simulink library "lib_SecCtrl_MASmsg"  (R2026a)
settings: Solver=VariableStepAuto
undefined symbols (not defined in the file): buses_lf, DiscIntNeverNeededParam, entity, iPs_lf, iQs_lf, last_send, m, Ps_lf, Qs_lf, set_DG_up, set_extra_satur, set_sending_cost, v_buses_mod
libraries: simulink x400, sl_discontinuities x10, eeGeneralControl x5
(part 4 of 12)

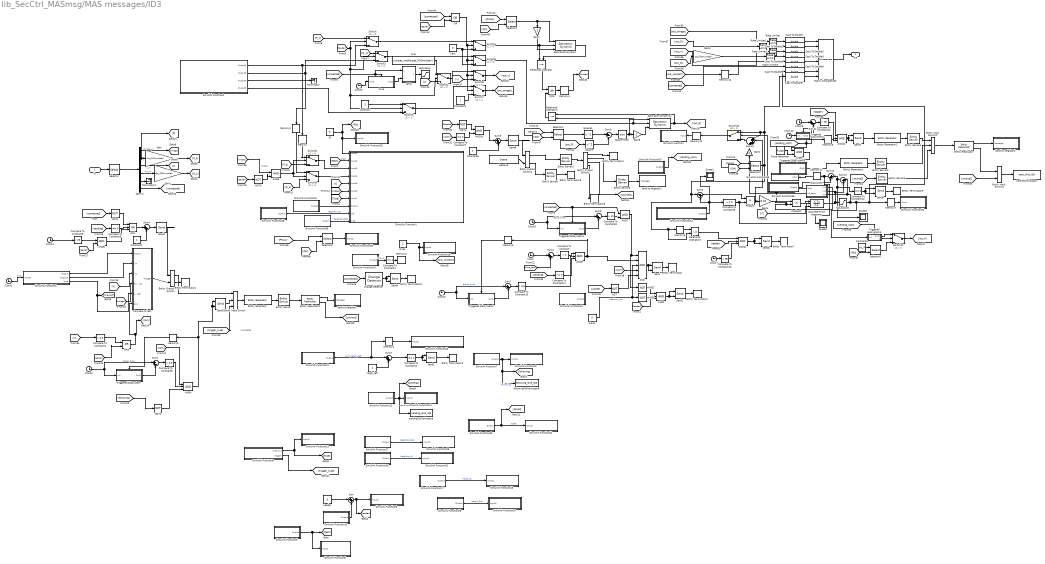
== system lib_SecCtrl_MASmsg/MAS messages/ID3 ==
  note: Variables
  in : Inport
  AND : Logic  Inputs=5  IconShape=distinctive  AllPortsSameDT=off  OutDataTypeStr=boolean
  AND{1,3..4,11..12} (5 alike) : Logic  Inputs=3  IconShape=distinctive  AllPortsSameDT=off  OutDataTypeStr=boolean
  AND{5..7,9..10} (5 alike) : Logic  IconShape=distinctive  AllPortsSameDT=off  OutDataTypeStr=boolean
  AND2 : Logic  Operator=NOT  IconShape=distinctive  AllPortsSameDT=off  OutDataTypeStr=boolean
  AND8 : Logic  Operator=NOT  IconShape=distinctive  AllPortsSameDT=off  OutDataTypeStr=boolean
  Cast To Double{,1..7} (8 alike) : DataTypeConversion  OutDataTypeStr=double  SaturateOnIntegerOverflow=off  RndMeth=Floor
  Change Detector : eeGeneralControl/Change Detector  VariantControl=Variant1  LabelModeActiveChoice=Discrete  ChangeType=Falling edge  x0=0  Ts=-1
  Clock{,1..8,10} (10 alike) : Clock
  Compare To Constant : simulink/Logic and Bit Operations/Compare To Constant  relop=>  const=2  OutDataTypeStr=boolean  ZeroCross=off
  Compare To Constant1 : simulink/Logic and Bit Operations/Compare To Constant  relop===  const=1  OutDataTypeStr=boolean  ZeroCross=off
  Compare To Constant10 : simulink/Logic and Bit Operations/Compare To Constant  relop=>  const=0.5  OutDataTypeStr=boolean  ZeroCross=off
  Compare To Constant11 : simulink/Logic and Bit Operations/Compare To Constant  relop=~=  const=0  OutDataTypeStr=uint8  ZeroCross=off
  Compare To Constant12 : simulink/Logic and Bit Operations/Compare To Constant  relop=>  const=90  OutDataTypeStr=boolean
  Compare To Constant13 : simulink/Logic and Bit Operations/Compare To Constant  relop=>  const=95  OutDataTypeStr=boolean
  Compare To Constant14 : simulink/Logic and Bit Operations/Compare To Constant  relop===  const=0  OutDataTypeStr=boolean
  Compare To Constant2 : simulink/Logic and Bit Operations/Compare To Constant  relop===  const=0  OutDataTypeStr=boolean  ZeroCross=off
  Compare To Constant3 : simulink/Logic and Bit Operations/Compare To Constant  relop===  const=0  OutDataTypeStr=uint8  ZeroCross=off
  Compare To Constant4 : simulink/Logic and Bit Operations/Compare To Constant  relop=>  const=0.5  OutDataTypeStr=boolean  ZeroCross=off
  Compare To Constant5 : simulink/Logic and Bit Operations/Compare To Constant  relop=>  const=0.5  OutDataTypeStr=boolean  ZeroCross=off
  Compare To Constant6 : simulink/Logic and Bit Operations/Compare To Constant  relop=<  const=25  OutDataTypeStr=boolean  ZeroCross=off
  Compare To Constant7 : simulink/Logic and Bit Operations/Compare To Constant  relop===  const=0  OutDataTypeStr=uint8  ZeroCross=off
  Compare To Constant8 : simulink/Logic and Bit Operations/Compare To Constant  relop=>  const=10  OutDataTypeStr=boolean  ZeroCross=off
  Compare To Constant9 : simulink/Logic and Bit Operations/Compare To Constant  relop=~=  const=0  OutDataTypeStr=boolean
  Compare to last : Subsystem
  Constant{,1..2,6} (4 alike) : Constant
  Constant3 : Constant  Value=Ps_lf  VectorParams1D=off
  Demux : Demux  Outputs=6
  Discrete-Time Integrator : DiscreteIntegrator  ExternalReset=rising  InitialConditionSource=external  ICPrevOutput=DiscIntNeverNeededParam  ICPrevScaledInput=DiscIntNeverNeededParam
  Entity Input Switch : EntityInputSwitch  InputPortMessageModes=m,m,m  OutputPortMessageModes=m  NumberInputPorts=3
      settings: InputPortMap=u1,u2,u3
  Entity Input Switch1 : EntityInputSwitch  InputPortMessageModes=m,m  OutputPortMessageModes=m
  Entity Input Switch2 : EntityInputSwitch  InputPortMessageModes=m,m,m  OutputPortMessageModes=m  NumberInputPorts=3
      settings: InputPortMap=u1,u2,u3
  Entity Output Switch : EntityOutputSwitch  InputPortMessageModes=m,m  OutputPortMessageModes=m,m  SwitchingCriterion=From control port  SwitchAttributeName=Attribute1
      settings: InputPortMap=u0,u1
  Entity Output Switch1 : EntityOutputSwitch  InputPortMessageModes=m,m  OutputPortMessageModes=m,m  SwitchingCriterion=From control port  SwitchAttributeName=Attribute1
      settings: InputPortMap=u0,u1
  Entity Output Switch2 : EntityOutputSwitch  InputPortMessageModes=m  OutputPortMessageModes=m,m,m,m  NumberOutputPorts=4  SwitchingCriterion=From attribute  SwitchAttributeName=Select
      settings: OutputPortMap=o0,o1,o2,o3
  Entity Generator : EntityGenerator  InputPortMessageModes=m  OutputPortMessageModes=m  GenerationMethod=Event-based  Period=0.01  AttributeName=DG_up|Source|Dest|P_s|Q_s|v|omega|Opt|type|Select|Neighbor_ID|Neighbor_Opt  AttributeInitialValue=0|0|0|0|0|0|0|1|0|0|1|1  EntityType=Structured  EntityTypeName=Message
      settings: InputPortMap=u0
  Entity Generator1 : EntityGenerator  InputPortMessageModes=m  OutputPortMessageModes=m  GenerationMethod=Event-based  TimeSource=Signal port  Period=0.1  GenerateEntityAtSimulationStart=off  AttributeName=DG_up|Source|Dest|P_s|Q_s|v|omega|Opt|type|Select|Neighbor_ID|Neighbor_Opt  AttributeInitialValue=0|0|0|0|0|0|0|1|0|0|1|1  EntityType=Structured  EntityTypeName=Message
      settings: InputPortMap=u0
  Entity Generator2 : EntityGenerator  InputPortMessageModes=m  OutputPortMessageModes=m  GenerationMethod=Event-based  TimeSource=Signal port  Period=0.1  GenerateEntityAtSimulationStart=off  AttributeName=DG_up|Source|Dest|P_s|Q_s|v|omega|Opt|type|Select|Neighbor_ID|Neighbor_Opt  AttributeInitialValue=0|0|0|0|0|0|0|1|0|0|1|1  EntityType=Structured  EntityTypeName=Message
      settings: InputPortMap=u0
  Entity Replicator : EntityReplicator  InputPortMessageModes=m  OutputPortMessageModes=m,m
  Entity Replicator1 : EntityReplicator  InputPortMessageModes=m  OutputPortMessageModes=m,m
  Entity Server : EntityServer  InputPortMessageModes=m  OutputPortMessageModes=m  Capacity=1  ServiceTimeValue=0.1  EntryAction=|  ServiceCompleteAction=last_send(entity.v, entity.omega);
      | [entity.Source, entity.Dest, entity.P_s, ...
      |     entity.Q_s, entity.v, entity.omega, ...
      |     entity.type, entity.Opt, entity.Neighbor_ID, ...
      |     entity.Neighbor_Opt] = package();
      | if entity.type == 0
      |     entity.Dest = get_following;
      | end
      | type(0);
      | send_to(0);
      | set_Neighbor_ID(0);
  Entity Server1 : EntityServer  InputPortMessageModes=m  OutputPortMessageModes=m  Capacity=1  ServiceTimeValue=1e-10
  Entity Server2 : EntityServer  InputPortMessageModes=m  OutputPortMessageModes=m  Capacity=1  ServiceTimeValue=1e-10  ServiceCompleteAction=|
      | if (entity.type == 0 & ...
      |         entity.Dest == get_ID & ...
      |         get_DG_up == 0 & get_sending ~= 0) ...
      |         | (entity.type == 8 & ...
      |         get_neigh_ID ~= get_ID)
      |     entity.Select = 2;
      |     entity.Source = get_ID;
      |     if entity.type == 8
      |         entity.Dest = get_neigh_ID;
      |     else
      |         entity.Dest = get_sending;
      |     end
      | elseif entity.type == 10
      |     entity.Dest = get_sending;
      |     if get_leader == 0
      |         set_sending_cost(0);
      |         entity.Select = 3;
      |     else
      |         set_sending_cost(0);
      |         set_cost_info(0);
      |         entity.Select = 4;
      |     end
      |     
      | else
      |     entity.Select = 1;
      | end
  Entity Server3 : EntityServer  InputPortMessageModes=m  OutputPortMessageModes=m  Capacity=1  ServiceTimeValue=0.05  EntryAction=|
      | aux = get_extra_satur();
      | if aux == 0
      |     entity.Opt = get_cost();
      | else
      |     entity.Opt = get_cost() + 100*aux;
      |     set_extra_satur(aux)
      | end
      | entity.P_s = get_cost_P();
      | entity.type = 9;
      | entity.Dest = get_sending();
      | entity.Source = get_ID();
  Entity Server4 : EntityServer  InputPortMessageModes=m  OutputPortMessageModes=m  Capacity=1  ServiceTimeValue=0.05  EntryAction=|
      | entity.type = 10;
      | entity.Dest = get_sending();
      | set_sending_cost(0)
      | set_cost_info(0)
      | entity.Source = get_ID();
  Entity Server5 : EntityServer  InputPortMessageModes=m  OutputPortMessageModes=m  Capacity=1  ServiceTimeValue=0.05  EntryAction=|
      | set_cost_info(0)
      | set_sending_cost(0)
      | entity.Source = get_ID();
  Entity Server6 : EntityServer  InputPortMessageModes=m  OutputPortMessageModes=m  Capacity=1  ServiceTimeValue=0.05
  Entity Terminator : EntityTerminator  InputPortMessageModes=m  EntryAction=|
      | set_Neighbor_Opt(get_ID);
      | set_original_Opt(get_ID);
      | set_Neighbor_ID(get_ID);
      | set_asked(1);
      | if get_DG_up
      |     optim_value = -5;
      | else
      |     optim_value = get_Opt();
      | end
      | if optim_value > get_neigh_Opt()
      |     set_neigh_ID(get_ID);
      |     set_neigh_Opt(optim_value);
      | end
      | type(6); % Startup?
  Entity Terminator1 : EntityTerminator  InputPortMessageModes=m  EntryAction=|
      | type_value = entity.type;
      | if get_leader == 0 % If I am not the leader  
      |     switch type_value
      |         case 0
      |             if entity.Dest == 0 & get_sending == 0 % New DG & I am free
      |                 if get_following() ~= 0 % If I follow someone
      |                     send_to(entity.Source); % Answer
      |                     type(1); % Follow me
      |                 end
      |             else
      |                 unpackage(entity.P_s,entity.Q_s,1,entity.omega);
      |             end
      |         case 1 % Wants follower
      |             if get_following() == 0 % No following
      |                 if get_sending ~= entity.Source % It does not follow me
      |                     send_to(entity.Source);
      |                     set_following(entity.Source);
      |                     type(2); % I follow you
      |                 end
      |             end
      |         case 2
      |             if get_following ~= entity.Source % I do not follow it
      |                 if get_following ~= 0 % If I follow someone
      |                     set_sending(entity.Source);
      |                 else
      |                     send_to(entity.Source);
      |                     type(5);
      |                 end
      |             else
      |                 set_following(0);
      |             end
      |         case 3
      |             if get_following ~= 0 & get_following ~= entity.Source % Following other
      |                 send_to(get_following);
      |                 set_following(0); % Exit following other
      |                 type(4); % I will not follow you
      |             else
      |                 send_to(entity.Source);
      |                 set_following(entity.Source);
      |                 type(2); % I follow you
      |             end
      |         case 4 % It will no longer follow me
      |             set_sending(0); % I am not sending
      |        case 5
      |            if get_following == entity.Source
      |                 set_following(0);
      |                 if get_sending ~= 0
      |                     send_to(get_sending);
      |                     type(5);
      |                     set_sending(0);
      |                 end
      |            end
      |         case 6 % startup?
      |             set_Neighbor_Opt(entity.Neighbor_Opt);
      |             if get_asked % If I asked
      |                 send_to(entity.Source);
      |                 set_Opt(-5);
      |                 type(7); % startup_data
      |             else % ask neighbors
      |                 if get_DG_up
      |                     optim_value = -5;
      |                 else
      |                     optim_value = get_Opt();
      |                 end
      |                 if optim_value > get_neigh_Opt()
      |                     set_neigh_ID(get_ID);
      |                     set_neigh_Opt(optim_value);
      |                 end
      |                 if entity.Neighbor_Opt ~= 0
      |                     set_original_Opt(entity.Neighbor_Opt);
      |                 end
      |                 set_original_ID(entity.Source);
      |                 set_asked(1);
      |                 send_to(0);
      |                 set_Neighbor_ID(get_ID);
      |                 type(6);
      |             end                 
      |         case 7 % startup_data
      |             set_sum_neigh_left(get_sum_neigh_left() - 1);
      |             if entity.Opt > get_neigh_Opt() % If this DG is better
      |                 set_neigh_ID(entity.Source);
      |                 set_neigh_Opt(entity.Opt);
      |             end
      |         case 8 % startup
      |             if ~get_DG_up()
      |                 set_DG_up(1);
      |                 if get_neigh_ID() == get_ID()
      |                     set_neigh_Opt(-5);
      |                 end
      |                 set_decision_turn(1);
      |                 unpackage(entity.P_s,entity.Q_s,1,entity.omega);
      |             end
      |         case 9 % cost and P info
      |             set_sending_cost(1)
      |             set_cost_info(entity.Opt)
      |     end
      |     if get_following() == 0 % No following
      |         [~,~,P_s,Q_s,v,omega,~] = package();
      |         unpackage(P_s, Q_s, v, omega);
      |     end
      | elseif get_leader() == 1 % If I am the leader
      |         if get_sending == 0 % If I have no followers
      |             if type_value == 2 % It follows me
      |                 set_sending(entity.Source);
      |             elseif type_value == 0 % New DG
      |                 type(3); % I am the leader, follow me
      |             end
      |         elseif type_value == 2
      |             if get_sending ~= entity.Source
      |                 send_to(entity.Source);
      |                 type(5);
      |             end
      |         elseif type_value == 1
      |             if get_following() == 0 % No following
      |                 if get_sending ~= entity.Source % It does not follow me
      |                     send_to(entity.Source);
      |                     set_following(entity.Source);
      |                     type(2); % I follow you
      |                 end
      |             end
      |         end
      |         if type_value == 6
      |             if get_asked % If I asked
      |                 send_to(entity.Source);
      |                 set_Opt(-5);
      |                 type(7); % startup_data
      |             else % ask neighbors
      |                 if get_DG_up
      |                     optim_value = -5;
      |                 else
      |                     optim_value = rand;
      |                 end
      |                 if optim_value > get_neigh_Opt()
      |                     set_neigh_ID(get_ID);
      |                     set_neigh_Opt(optim_value);
      |                 end
      |                 if entity.Neighbor_Opt ~= 0
      |                     set_original_Opt(entity.Neighbor_Opt);
      |                 end
      |                 set_original_ID(entity.Source);
      |                 set_asked(1);
      |                 send_to(0);
      |                 set_Neighbor_ID(get_ID);
      |                 set_Neighbor_Opt(entity.Neighbor_Opt);
      |                 type(6);
      |             end                 
      |         end
      |         if type_value == 7 % startup_data
      |             set_sum_neigh_left(get_sum_neigh_left()-1);
      |             if entity.Opt > get_neigh_Opt() % If this DG is better
      |                 set_neigh_ID(entity.Source);
      |                 set_neigh_Opt(entity.Opt);
      |             end
      |         end
      |         if type_value == 9 % cost and P info
      |             set_cost_info(entity.Opt)
      |         end
      | end
  Entity Terminator2 : EntityTerminator  InputPortMessageModes=m  EntryAction=|
      | set_DG_up(1);
      | set_decision_turn(1);
  Entity Terminator3 : EntityTerminator  InputPortMessageModes=m  EntryAction=|
      | set_sum_neigh_left(0);
      | set_asked(0);
      | if get_original_Opt == get_ID & get_neigh_ID ~= 0
      |     if get_ID ~= get_neigh_ID & get_neigh_Opt ~= -5
      |         send_to(get_neigh_ID);
      |         set_decision_turn(0);
      |         set_neigh_Opt(-10);
      |         type(8); % startup
      |     else
      |         if get_neigh_Opt == -5
      |             set_asked(0);
      |         end
      |     end
      | else
      |     set_Neighbor_ID(get_neigh_ID);
      |     set_Opt(get_neigh_Opt);
      |     set_Neighbor_Opt(get_original_Opt);
      |     send_to(get_original_ID);
      |     set_neigh_Opt(-10);
      |     type(7); % startup data
      | end
  Entity Terminator4 : EntityTerminator  InputPortMessageModes=m  EntryAction=|
      | [~, ~, ~, ~, v, omega, ~, ~, ~, ~] = package();
      | last_send(0,0);
  Entity Terminator5 : EntityTerminator  InputPortMessageModes=m  EntryAction=set_DG_up(0);
  Entity Terminator6 : EntityTerminator  InputPortMessageModes=m  EntryAction=|
      | if entity.type == 6 % asking for startup
      |     set_Opt(-5); % I cannot start
      |     send_to(entity.Source);
      |     type(7); % startup data
      | end
  Entity Terminator7 : EntityTerminator  InputPortMessageModes=m  EntryAction=set_sending_cost(1)
  Entity Terminator8 : EntityTerminator  InputPortMessageModes=m
  Entity Terminator9 : EntityTerminator  InputPortMessageModes=m  EntryAction=set_extra_satur(0)
  Gain : Gain  Gain=iPs_lf(IDnumber)
  Gain1 : Gain  Gain=iQs_lf(IDnumber)
  Gain2 : Gain  Gain=0.1
  Gain3 : Gain  Gain=Qs_lf(IDnumber)
  Gain4 : Gain  Gain=0.01
  Gain7 : Gain  Gain=-1
  Gain8 : Gain  Gain=-1
  ID : Constant  Value=3
  Leader : Constant  Value=0
  Matrix Concatenate : Concatenate  NumInputs=8  Mode=Multidimensional array
  Memory{,1,3..11} (11 alike) : Memory
  Memory12 : Memory  InitialCondition=1
  Memory2 : Memory  InitialCondition=1
  NOT{,1..4} (5 alike) : Logic  Operator=NOT  IconShape=distinctive  AllPortsSameDT=off  OutDataTypeStr=boolean
  OR : Logic  Operator=OR  IconShape=distinctive  AllPortsSameDT=off  OutDataTypeStr=boolean
  OR1 : Logic  Operator=OR  Inputs=3  IconShape=distinctive  AllPortsSameDT=off  OutDataTypeStr=boolean
  OR2 : Logic  Operator=OR  IconShape=distinctive  AllPortsSameDT=off  OutDataTypeStr=boolean
  OR3 : Logic  Operator=OR  IconShape=distinctive  AllPortsSameDT=off  OutDataTypeStr=boolean
  One : Constant  Value=v_buses_mod(buses_lf(IDnumber))  OutDataTypeStr=Inherit: Inherit via back propagation
  One1 : Constant  OutDataTypeStr=Inherit: Inherit via back propagation
  Product : Product
  Product1 : Product
  Pulse Generator : DiscretePulseGenerator  PulseType=Time based  Period=1  PulseWidth=50  PhaseDelay=0.5
  Rate Limiter : RateLimiter  RisingSlewLimit=0.1  FallingSlewLimit=-0.1  SampleTimeMode=inherited  InitialCondition=1
  Rate Limiter1 : RateLimiter  RisingSlewLimit=0.1  FallingSlewLimit=-0.1  SampleTimeMode=inherited  InitialCondition=Ps_lf(IDnumber)
  Rate Limiter2 : RateLimiter  RisingSlewLimit=0.1  FallingSlewLimit=-0.1  SampleTimeMode=inherited  InitialCondition=v_buses_mod(buses_lf(IDnumber))
  Rate Limiter3 : RateLimiter  RisingSlewLimit=0.1  FallingSlewLimit=-0.1  SampleTimeMode=inherited  InitialCondition=Qs_lf(IDnumber)
  Receive : Queue  OutputPortMessageModes=m  Capacity=10  EntityArrivalSource=Multicast  MulticastTag=ID3
  Relational Operator : RelationalOperator  Operator=~=  OutDataTypeStr=boolean  ZeroCross=off  RndMeth=Simplest  InputSameDT=off
  Relational Operator1 : RelationalOperator  Operator=~=  OutDataTypeStr=boolean  ZeroCross=off  RndMeth=Simplest  InputSameDT=off
  Relational Operator2 : RelationalOperator  Operator=~=  OutDataTypeStr=boolean  RndMeth=Simplest  InputSameDT=off
  Saturation : Saturate  UpperLimit=1  LowerLimit=0  ZeroCross=off
  Saturation Dynamic : sl_discontinuities/Saturation Dynamic  OutMin=[]  OutMax=[]  OutDataTypeStr=Inherit: Same as second input  OutDataType=fixdt(1, 16)  OutScaling=2^-10  DoSatur=off
  Saturation Dynamic1 : sl_discontinuities/Saturation Dynamic  OutMin=[]  OutMax=[]  OutDataTypeStr=Inherit: Same as second input  OutDataType=fixdt(1, 16)  OutScaling=2^-10  DoSatur=off
  Saturation1 : Saturate  UpperLimit=6  LowerLimit=0.1
  Scope1 : Scope
      settings: ActiveDisplayYMinimum=-0.38013  ActiveDisplayYMaximum=3.4211  DataLoggingVariableName=ScopeData2
  Scope2 : Scope
      settings: ActiveDisplayYMinimum=-6.8507  ActiveDisplayYMaximum=6.8507
  Scope3 : Scope
      settings: ActiveDisplayYMinimum=-0.0007  ActiveDisplayYMaximum=0.00633  DataLoggingVariableName=ScopeData2
  Selector : Selector  NumberOfDimensions=2  InputPortWidth=3  IndexOptions=Select all,Index vector (dialog)  Indices=ID,str2double(ID)  OutputSizes=1,1
  Selector{1..5} (5 alike) : Selector  InputPortWidth=length(buses_lf)  IndexOptions=Index vector (port)  Indices=[1 3]  OutputSizes=1
  Send{,1..2,4..5,7..9} (8 alike) : Send  OutputPortMessageModes=m  ShowEnablePort=on
      settings: InputPortMap=e0,u1
  Send to neighbor : Subsystem  Variant=on  VariantControlMode=label  LabelModeActiveChoice=two  mask(Send_to_neighbor){}
  Send to neighbor1 : Subsystem  Variant=on  VariantControlMode=label  LabelModeActiveChoice=two  mask(Send_to_neighbor){}
  Send to neighbor2 : Subsystem  Variant=on  VariantControlMode=label  LabelModeActiveChoice=two  mask(Send_to_neighbor){}
  Send3 : Send  OutputPortMessageModes=m
  Send6 : Send  OutputPortMessageModes=m
  Simulink Function : Subsystem  TreatAsAtomicUnit=on
  Simulink Function1 : Subsystem  TreatAsAtomicUnit=on
  Simulink Function10 : Subsystem  TreatAsAtomicUnit=on
  Simulink Function11 : Subsystem  TreatAsAtomicUnit=on
  Simulink Function12 : Subsystem  TreatAsAtomicUnit=on
  Simulink Function13 : Subsystem  TreatAsAtomicUnit=on
  Simulink Function14 : Subsystem  TreatAsAtomicUnit=on
  Simulink Function15 : Subsystem  TreatAsAtomicUnit=on
  Simulink Function16 : Subsystem  TreatAsAtomicUnit=on
  Simulink Function17 : Subsystem  TreatAsAtomicUnit=on
  Simulink Function18 : Subsystem  TreatAsAtomicUnit=on
  Simulink Function19 : Subsystem  TreatAsAtomicUnit=on
  Simulink Function2 : Subsystem  TreatAsAtomicUnit=on
  Simulink Function20 : Subsystem  TreatAsAtomicUnit=on
  Simulink Function21 : Subsystem  TreatAsAtomicUnit=on
  Simulink Function22 : Subsystem  TreatAsAtomicUnit=on
  Simulink Function23 : Subsystem  TreatAsAtomicUnit=on
  Simulink Function24 : Subsystem  TreatAsAtomicUnit=on
  Simulink Function25 : Subsystem  TreatAsAtomicUnit=on
  Simulink Function26 : Subsystem  TreatAsAtomicUnit=on
  Simulink Function27 : Subsystem  TreatAsAtomicUnit=on
  Simulink Function28 : Subsystem  TreatAsAtomicUnit=on
  Simulink Function29 : Subsystem  TreatAsAtomicUnit=on
  Simulink Function3 : Subsystem  TreatAsAtomicUnit=on
  Simulink Function30 : Subsystem  TreatAsAtomicUnit=on
  Simulink Function31 : Subsystem  TreatAsAtomicUnit=on
  Simulink Function32 : Subsystem  TreatAsAtomicUnit=on
  Simulink Function33 : Subsystem  TreatAsAtomicUnit=on
  Simulink Function34 : Subsystem  TreatAsAtomicUnit=on
  Simulink Function35 : Subsystem  TreatAsAtomicUnit=on
  Simulink Function36 : Subsystem  TreatAsAtomicUnit=on
  Simulink Function37 : Subsystem  TreatAsAtomicUnit=on
  Simulink Function38 : Subsystem  TreatAsAtomicUnit=on
  Simulink Function4 : Subsystem  TreatAsAtomicUnit=on
  Simulink Function5 : Subsystem  TreatAsAtomicUnit=on
  Simulink Function6 : Subsystem  TreatAsAtomicUnit=on
  Simulink Function7 : Subsystem  TreatAsAtomicUnit=on
  Simulink Function8 : Subsystem  TreatAsAtomicUnit=on
  Simulink Function9 : Subsystem  TreatAsAtomicUnit=on
  Square : Math  Operator=square
  Square Root : Sqrt
  Square1 : Math  Operator=square
  Subsystem : Subsystem
  Sum{,2..4,6} (5 alike) : Sum  Inputs=|++
  Sum{1,5,7..8,11..12} (6 alike) : Sum  Inputs=|+-
  Sum10 : Sum  Inputs=|-+
  Sum13 : Sum  Inputs=|++++
  Sum9 : Sum  Inputs=|-+
  Switch{,1..9} (10 alike) : Switch  Criteria=u2 > Threshold  ZeroCross=off  SaturateOnIntegerOverflow=off  InputSameDT=off
  Switch10 : Switch  Criteria=u2 > Threshold  SaturateOnIntegerOverflow=off  InputSameDT=off
  Switch11 : Switch  Criteria=u2 > Threshold  SaturateOnIntegerOverflow=off  InputSameDT=off
  Terminator : Terminator
  Terminator1 : Terminator
  Triggered Subsystem : Subsystem  TreatAsAtomicUnit=on
  Triggered Subsystem1 : Subsystem  TreatAsAtomicUnit=on
  Triggered Subsystem2 : Subsystem  TreatAsAtomicUnit=on
  Triggered Subsystem3 : Subsystem  TreatAsAtomicUnit=on
  Triggered Subsystem4 : Subsystem  TreatAsAtomicUnit=on
  Triggered Subsystem5 : Subsystem  TreatAsAtomicUnit=on
  Zero : Constant  Value=0  OutDataTypeStr=Inherit: Inherit via back propagation
  Zero1 : Constant  Value=0  OutDataTypeStr=Inherit: Inherit via back propagation
  followingToWorkspace : ToWorkspace  VariableName=following_Grid_ID3  SampleTime=-1
      settings: MaxDataPoints=1
  neigh_left : Constant  Value=2
  ramp : Subsystem
  sendingToWorkspace : ToWorkspace  VariableName=sending_Grid_ID3  SampleTime=-1
      settings: MaxDataPoints=1
  sentToWorkspace : ToWorkspace  VariableName=sent_Grid_ID3  SaveFormat=Timeseries  SampleTime=-1
  time : Subsystem  TreatAsAtomicUnit=on
  out : Outport
  wires:
  [IDn] -> Selector2/2
  [Snom] -> Selector2/1
  [IDn] -> Selector1/2
  Selector1/1 -> Gain7/1, Saturation Dynamic/1
  Square Root/1 -> Gain8/1, Saturation Dynamic1/1
  Square1/1 -> Sum5/1
  Sum5/1 -> Square Root/1
  Square/1 -> Sum5/2
  Selector2/1 -> Square1/1
  [out_P] -> Square/1
  Cast To Double5/1 -> Matrix Concatenate/6
  Cast To Double4/1 -> Matrix Concatenate/5
  Cast To Double3/1 -> Matrix Concatenate/4
  Cast To Double2/1 -> Matrix Concatenate/3
  Cast To Double1/1 -> Matrix Concatenate/2
  Cast To Double/1 -> Matrix Concatenate/1
  Entity Output Switch2/2 -> Entity Server6/1
  Selector/1 -> Demux/1
  Demux/2 -> [P], Gain/1
  Demux/6 -> [connected]
  Demux/5 -> Terminator1/1
  in/1 -> Selector/1
  [connected] -> OR/1
  [connected] -> Cast To Double5/1
  [out_connect] -> Memory12/1
  Matrix Concatenate/1 -> out/1
  [out_Q] -> Gain3/1
  [out_v] -> Rate Limiter2/1
  [out_omega] -> Rate Limiter/1
  Switch7/1 -> [out_omega]
  Compare To Constant11/1 -> AND3/3
  [sending] -> Compare To Constant11/1
  Memory6/1 -> Triggered Subsystem2/Trigger
  Compare To Constant10/1 -> AND3/2
  Compare To Constant/1 -> AND3/1
  AND3/1 -> AND/2, Memory6/1
  Clock3/1 -> Sum7/1, Triggered Subsystem2/1(In1)  "actual_time"
  Triggered Subsystem2/1(Out1) -> Sum7/2
  Sum7/1 -> Compare To Constant10/1
  Sum2/1 -> Compare To Constant/1
  Clock/1 -> Sum2/1
  [time_last] -> Sum2/2
  Memory5/1 -> Triggered Subsystem/Trigger
  Triggered Subsystem/1(Out1) -> Sum1/2
  Entity Server1/1 -> Entity Terminator6/1
  [leader] -> OR2/2
  Compare To Constant4/1 -> OR2/1
  [com] -> AND4/1
  Compare To Constant7/1 -> AND10/2
  NOT4/1 -> AND10/1
  [leader] -> NOT4/1
  Constant6/1 -> Sum6/2
  AND10/1 -> Sum6/1
  [com] -> Compare To Constant7/1
  Send6/1 -> Entity Output Switch1/1
  Sum6/1 -> Send6/1
  Entity Output Switch1/2 -> Entity Server1/1
  [com] -> AND/4
  AND8/1 -> AND1/3
  AND7/1 -> AND2/1, AND/1
  Clock5/1 -> time/1(time)
  time/1(Out1) -> ramp/2(time)
  ramp/1(Out1) -> Saturation/1
  [connected] -> time/Trigger, ramp/1(connected)
  [v] -> Compare To Constant4/1
  OR2/1 -> [com], Compare to last/6(com)
  [trigger_type] -> Entity Input Switch/3
  Compare To Constant5/1 -> AND4/2
  Simulink Function8/2(trigger) -> [trigger_type]
  Switch6/1 -> [out_v]
  Relational Operator1/1 -> OR3/2
  OR3/1 -> Memory4/1
  Memory4/1 -> [limited]
  Switch4/1 -> Saturation Dynamic/2, Relational Operator/1
  Gain7/1 -> Saturation Dynamic/3
  Gain8/1 -> Saturation Dynamic1/3
  [Pmax] -> Selector1/1
  Saturation Dynamic1/1 -> Relational Operator1/1, [out_Q]
  Switch5/1 -> Saturation Dynamic1/2, Relational Operator1/2
  Relational Operator/1 -> OR3/1
  Saturation Dynamic/1 -> Relational Operator/2
  AND6/1 -> Switch8/2, Switch9/2
  [limited] -> AND6/1  "limited"
  NOT3/1 -> AND6/2
  [leader] -> NOT3/1
  Memory3/1 -> Switch9/1
  Memory/1 -> Switch8/1
  Switch9/1 -> Simulink Function1/4(Input4)
  Switch8/1 -> Simulink Function1/3(Input3)
  [Q_s] -> Switch9/3
  [P_s] -> Switch8/3
  Compare To Constant1/1 -> Memory2/1
  Send4/1 -> Entity Terminator5/1
  Change Detector/1 -> Send4/2, Send4/1
  [connected] -> Change Detector/1
  Simulink Function15/1(Output) -> Compare To Constant1/1  "DG_up"
  Clock4/1 -> Compare To Constant6/1
  [leader] -> AND5/2
  Compare To Constant6/1 -> AND5/1
  AND5/1 -> OR1/3
  NOT1/1 -> OR1/1
  [Pmax] -> Selector3/1
  One1/1 -> [out_connect], Simulink Function16/1(Input1)
  Entity Output Switch2/1 -> Entity Terminator1/1
  Entity Output Switch1/1 -> Entity Server2/1
  Clock2/1 -> Triggered Subsystem/1(In1), Sum1/1  "actual_time"
  Sum1/1 -> Compare To Constant5/1
  [following] -> NOT2/1
  NOT/1 -> AND/5
  [asked] -> NOT/1
  Simulink Function32/1(Output) -> Simulink Function34/1(Input1), [asked]  "asked"
  AND4/1 -> Send5/1, Send5/2, Memory5/1
  Receive/1 -> Entity Output Switch1/2
  Entity Server2/1 -> Entity Output Switch2/1
  [connected] -> NOT1/1
  OR1/1 -> Sum4/1
  Compare To Constant3/1 -> OR1/2
  Simulink Function30/1(Output) -> Simulink Function31/1(Input1)  "Neighbor_ID"
  Simulink Function27/1(Output) -> Simulink Function29/1(Input1)  "Neighbor_Opt"
  Entity Generator/1 -> Entity Server/1
  Simulink Function28/1(Output) -> Simulink Function1/10(In10)  "Neighbor_Opt"
  Simulink Function26/1(Output) -> Simulink Function1/9(In9)  "Neighbor_ID"
  [v] -> Switch6/3
  Zero/1 -> Switch4/3, Switch5/3
  Switch3/1 -> Switch7/1
  Switch2/1 -> Switch6/1
  Switch1/1 -> Switch5/1
  Switch/1 -> Switch4/1
  [leader] -> OR/2
  Constant2/1 -> Switch7/3
  OR/1 -> Switch4/2, Switch5/2, Switch6/2, Switch7/2
  Simulink Function4/1(Output) -> Compare to last/1(Output)
  Simulink Function4/2(Output1) -> Compare to last/2(In4)
  [omega] -> Compare to last/4(Output1)
  [v] -> Compare to last/3(In1)
  [v] -> Switch2/3
  Sum4/1 -> Send3/1
  Compare to last/1(Trigger) -> Entity Output Switch/2
  Entity Output Switch/2 -> Entity Terminator4/1
  Constant1/1 -> Sum4/2
  [sending] -> Compare To Constant3/1
  Send3/1 -> Entity Output Switch/1
  Memory1/1 -> Simulink Function23/1(Input1)
  Send2/1 -> Entity Terminator3/1
  Compare To Constant2/1 -> Send2/2, Send2/1
  Zero1/1 -> AND8/1, AND/3  "decision_turn"
  neigh_left/1 -> Sum3/2
  Sum3/1 -> Compare To Constant2/1
  Simulink Function21/1(Output) -> Sum3/1, Memory1/1  "sum_neigh_left"
  Simulink Function17/1(Output) -> Simulink Function18/1(Input1)  "neigh_ID"
  Simulink Function19/1(Output) -> Simulink Function20/1(Input1)  "neigh_Opt"
  Simulink Function22/1(Output) -> Simulink Function1/8(Output)
  Constant/1 -> Switch3/1
  [P_s] -> Switch/1
  [Q_s] -> Switch1/1
  Send1/1 -> Entity Terminator2/1
  AND1/1 -> Send1/2, Send1/1
  AND2/1 -> AND1/1
  [leader] -> AND1/2
  Send/1 -> Entity Terminator/1
  AND/1 -> Send/1, Send/2
  Clock1/1 -> Simulink Function4/1(Input2)  "time"
  Simulink Function4/3(time) -> [time_last], Compare to last/5(time_last)
  Entity Output Switch/1 -> Entity Input Switch/1
  [omega] -> Simulink Function1/6(Input5)
  [v] -> Simulink Function1/5(Input6)
  Send5/1 -> Entity Input Switch/2
  Simulink Function12/1(Output) -> Simulink Function11/1(Input1), sendingToWorkspace/1, [sending]  "sending"
  Simulink Function7/1(Output) -> Simulink Function3/1(Input1), [following], followingToWorkspace/1  "following"
  Simulink Function10/1(Output) -> Sum/2
  Sum/1 -> Simulink Function9/1(Input1), [leader]
  Leader/1 -> Sum/1
  Entity Input Switch/1 -> Entity Generator/1
  Simulink Function8/1(type_out) -> Simulink Function13/1(Input1), [Type]
  ID/1 -> [IDn], Simulink Function25/1(Input1), Simulink Function1/1(Input1)
  [Type] -> Simulink Function1/7(Input7)
  Demux/4 -> Gain1/1  "Q_s_in"
  Demux/3 -> [v]  "v_in"
  Simulink Function5/1(Output) -> [Dest], Simulink Function6/1(Input1)
  [Dest] -> Simulink Function1/2(Input2)  "Dest"
  Demux/1 -> [omega]  "omega_in"
  Selector3/1 -> Simulink Function36/1(Input1)
  [IDn] -> Selector3/2
  Sum8/1 -> Compare To Constant8/1
  Triggered Subsystem1/1(Out1) -> Sum8/2
  Clock6/1 -> Triggered Subsystem1/1(In1), Sum8/1  "actual_time"
  [connected] -> AND7/1, Triggered Subsystem1/Trigger
  Compare To Constant8/1 -> AND7/2
  [leader] -> Switch/2, Switch1/2, Switch2/2, Switch3/2
  Simulink Function2/1(Output2) -> Switch/3, Memory/1
  Simulink Function2/2(Output3) -> Switch1/3, Memory3/1
  Simulink Function2/3(Output4) -> Terminator/1
  Simulink Function2/4(Output5) -> Switch3/3
  One/1 -> Switch2/1
  Gain/1 -> [P_s]
  Gain1/1 -> [Q_s]
  [out_P] -> Rate Limiter1/1
  Gain3/1 -> Rate Limiter3/1
  Rate Limiter/1 -> Cast To Double/1
  Rate Limiter1/1 -> Cast To Double1/1
  Rate Limiter2/1 -> Cast To Double2/1
  Rate Limiter3/1 -> Cast To Double3/1
  NOT2/1 -> AND4/3
  [costs] -> Selector4/1
  [IDn] -> Selector4/2
  Entity Generator2/1 -> Entity Server4/1
  Selector4/1 -> Relational Operator2/2, Memory8/1, Sum9/1, Cast To Double7/1, Sum13/1, Switch10/1
  Product/1 -> Sum13/2, Gain4/1
  Simulink Function14/1(Output) -> Scope1/1, Compare To Constant9/1, Sum9/2
  Compare To Constant9/1 -> Discrete-Time Integrator/2, Product/2
  Discrete-Time Integrator/1 -> Sum10/2, Subsystem/2(In3), Saturation1/1
  Memory7/1 -> Simulink Function33/1(Input)
  Gain4/1 -> Subsystem/1(In1), Product1/2
  Cast To Double7/1 -> Matrix Concatenate/8
  Cast To Double6/1 -> Matrix Concatenate/7
  Saturation1/1 -> Sum10/1, Subsystem/3(In4), Triggered Subsystem5/1(In1), Memory7/1, Cast To Double6/1
  Sum9/1 -> Product/1
  Triggered Subsystem3/1(Out1) -> Entity Generator1/1
  Sum12/1 -> Compare To Constant12/1
  Clock8/1 -> Sum12/1
  Compare To Constant12/1 -> AND12/2
  Send7/1 -> Entity Generator2/1
  Entity Generator1/1 -> Entity Server3/1
  Entity Server3/1 -> Entity Input Switch2/2
  Entity Server4/1 -> Entity Input Switch2/1
  Pulse Generator/1 -> AND9/2
  [sending_cost] -> Triggered Subsystem4/Trigger, Memory9/1, AND9/1
  AND9/1 -> Triggered Subsystem3/Trigger
  Simulink Function37/1(Output) -> [sending_cost]
  [leader] -> AND11/2
  [source1] -> Entity Input Switch1/2
  Entity Replicator/1 -> Send to neighbor2/1(Message)
  Entity Input Switch1/1 -> sentToWorkspace/1
  Entity Input Switch2/1 -> Entity Replicator/1
  Entity Replicator/2 -> Entity Input Switch1/1
  Entity Replicator1/2 -> [source1]
  Entity Server/1 -> Entity Replicator1/1
  Entity Replicator1/1 -> Send to neighbor/1(Message)
  AND12/1 -> Send7/1, Send7/2
  Memory9/1 -> AND12/3
  Clock10/1 -> Triggered Subsystem4/1(In1)
  Triggered Subsystem4/1(Out1) -> Sum12/2
  Entity Output Switch2/3 -> [source2]
  [source2] -> Entity Server5/1
  Entity Server5/1 -> Entity Input Switch2/3
  Sum13/1 -> Switch10/3
  Subsystem/1(Out1) -> Switch10/2, Product1/1
  AND11/1 -> Send8/1, Send8/2
  Send8/1 -> Entity Terminator7/1
  Memory8/1 -> Relational Operator2/1
  Compare To Constant13/1 -> AND11/3
  Clock7/1 -> Compare To Constant13/1
  Relational Operator2/1 -> AND11/1
  [leader] -> AND12/1
  Entity Output Switch2/4 -> Entity Terminator8/1
  [sending_cost] -> Triggered Subsystem5/Trigger
  Triggered Subsystem5/2(Output) -> Switch11/2
  Switch11/1 -> [out_P]
  [IDn] -> Selector5/2
  Constant3/1 -> Selector5/1
  Triggered Subsystem5/1(Out1) -> Switch11/1
  Selector5/1 -> Switch11/3
  Subsystem/2(inf_satur) -> Gain2/1
  Sum10/1 -> Scope3/1, Compare To Constant14/1, Sum11/1
  Simulink Function38/1(Output) -> Sum11/2
  Sum11/1 -> Scope2/1, Memory11/1
  Memory11/1 -> Simulink Function35/1(Input)
  Compare To Constant14/1 -> Send9/1, Send9/2
  Send9/1 -> Entity Terminator9/1
  Switch10/1 -> Memory10/1
  Memory10/1 -> Simulink Function/1(Input)
  Entity Server6/1 -> Send to neighbor1/1(Message)
  Product1/1 -> Discrete-Time Integrator/1
  [P] -> Discrete-Time Integrator/3
  Memory12/1 -> Cast To Double4/1
